simulink model "KinarmSimonTask_260119"  (R2019b)
settings: Solver=ode4  StartTime=0.0  StopTime=inf  FixedStep=BKIN_STEP_TIME  RelTol=1e-3  EnableMultiTasking=on
StartFcn:
  |  warndlg('Dexterit-E models cannot run under simulation. Please compile your model and run it from within Dexterit-E.');set_param(bdroot,'SimulationCommand','stop')
model workspace (MAT data in the model file):
  BKIN_KINEMATIC_FRAME_SIZE = 400
  BKIN_STEP_TIME = 0.00025
  E_COL_LSTIM = 8
  E_COL_RSTIM = 9
  E_CONG = 16
  E_CORRECT = 22
  E_FALSE_START = 28
  E_FIX_OFF = 11
  E_FIX_ON = 31
  E_INCONG = 17
  E_INCORRECT = 24
  E_LEFT_REACHED = 1
  E_LOC_LSIDE = 5
  E_LOC_NEUT = 7
  E_LOC_RSIDE = 6
  E_NEUTRAL = 10
  E_NO_EVENT = 0
  E_RIGHT_REACHED = 2
  E_STIM_OFF = 13
  E_STIM_ON = 12
  E_TIMED_OUT = 29
  E_TRIAL_END = 30
  E_TRIAL_START = 3
  E_WALLS_ON = 4
  FIX_OFF_TIME = 12
  FIX_ON_TIME = 11
  FIX_RAND = 13
  FIX_TARG_COL = 9
  FLICKER_ON = 9
  FLICKER_TIME = 10
  IMAGE_1 = 6
  IMAGE_2 = 7
  INST_TARG_COL = 1
  LBARR_TARG_COL = 4
  LENGTH = 3
  LOAD_X = 1
  LOAD_Y = 2
  LWALL_TARG_COL = 3
  NEUT_ON = 8
  PERTURB_SET = 10
  POSTRESP_DELAY = 4
  RADIUS_VIS = 3
  RBARR_TARG_COL = 6
  REACH_DELAY = 1
  REACH_RAND = 2
  REACH_TO = 3
  RESULT_TARG_COL = 8
  RWALL_TARG_COL = 5
  SPRING_CONST = 5
  START_BLOCK = 14
  START_TARG_COL = 2
  STIM_DIST = 6
  STIM_TARG_COL = 7
  STROKE_WIDTH = 10
  TARG_LENGTH = 3
  TARG_WIDTH = 4
  TEXT = 8
  TEXT_SIZE = 9
  WALL_SHAKE_TOGGLE = 7
  WIDTH = 4
  Width = 4
  X_LENGTH = 4
  Y_LENGTH = 5
  col_x = 1
  col_y = 2
undefined symbols (not defined in the file or in its folder): slselsubs
libraries: Video x11, General x3, KINARM_general x3, KINARM_EP_loads x2
settings Model: ModifiedComment=chris -- Wed Feb 16 09:18:30 2005 -- Version 1.1384  ModifiedHistory=Feb 16/05 - Add error repeat, add offset ramp  ExtModeArmWhenConnect=off  ExtModeLogAll=off  OrderedModelArguments=off  Creator=Chris Grebeldinger  LastModifiedBy=apark2
settings SolverCC: AutoInsertRateTranBlk=on
settings DataIOCC: SaveFormat=Array  SignalLoggingSaveFormat=ModelDataLogs  SaveOutput=off  SaveTime=off  ReturnWorkspaceOutputs=off  SignalLoggingName=sigsOut
settings OptimizationCC: BlockReduction=off  BooleanDataType=off  OptimizeBlockIOStorage=off  BufferReuse=off  GlobalBufferReuse=off  ExpressionFolding=off  ExpressionDepthLimit=2147483647  LocalBlockOutputs=off  InitFltsAndDblsToZero=on  LifeSpan=inf  OptimizeDataStoreBuffers=off  BusAssignmentInplaceUpdate=off
settings DebuggingCC: SaveWithParameterizedLinksMsg=none  UnderspecifiedInitializationDetection=Classic  MergeDetectMultiDrivingBlocksExec=none  SignalResolutionControl=TryResolveAllWithWarning  MultiTaskDSMMsg=warning  FcnCallInpInsideContextMsg=warning  BusObjectLabelMismatch=none  StateNameClashWarn=warning  StrictBusMsg=ErrorOnBusTreatedAsVector  SFUnexpectedBacktrackingDiag=warning  SFNoUnconditionalDefaultTransitionDiag=warning  SFExecutionAtInitializationDiag=none  ArithmeticOperatorsInVariantConditions=warning
settings HardwareCC: ProdBitPerPointer=32  ProdBitPerSizeT=32  ProdBitPerPtrDiffT=32  ProdLargestAtomicFloat=None  ProdWordSize=32  ProdLongLongMode=on  ProdHWDeviceType=Generic->32-bit x86 compatible  TargetLongLongMode=on  TargetIntDivRoundTo=Zero  TargetEndianess=LittleEndian  TargetHWDeviceType=Generic->32-bit x86 compatible
settings ModelReferenceCC: PropagateSignalLabelsOutOfModel=off
settings SFSimCC: SimCustomHeaderCode="#include \"stdlib.h\""  SimUseLocalCustomCode=off  SimParseCustomCode=off  CustomCodeUndefinedFunction=UseInterfaceOnly
settings RTWCC: Description=Simulink Real-Time  SystemTargetFile=slrt.tlc  TemplateMakefile=slrt_default_tmf  RTWUseLocalCustomCode=off  CustomSourceCode="#include \"stdlib.h\""  CodeExecutionProfiling=on
settings CodeAppCC: MaxIdLength=63  StateflowObjectComments=on
settings SimulinkRealTimeCC: TargetFcnLib=ansi_tfl_tmw.mat  GeneratePreprocessorConditionals=Disable all  PreserveStateflowLocalDataDimensions=off
settings ConfigComp: CovMetricSettings=dw  CovHtmlReporting=on  CovSaveCumulativeToWorkspaceVar=on  CovSaveSingleToWorkspaceVar=on  CovExternalEMLEnable=off

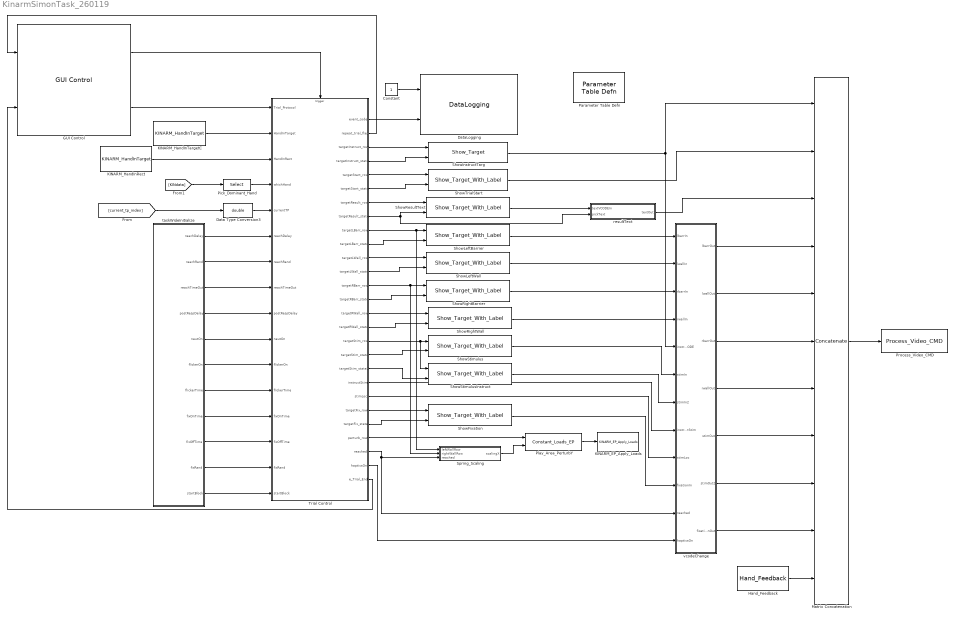
== system KinarmSimonTask_260119 ==
  Constant : Constant
  Data Type Conversion3 : DataTypeConversion  OutDataTypeStr=double
  DataLogging : General/DataLogging  log_event_codes=on  log_analog_inputs=off  show_time_remaining=off  ecat_include=on
  GUI Control : General/GUI Control  task_version=1.0  show_repeat_trial_flag=on  use_custom_tp=off  target_type_str=Circle  Target_Type=1  XYcols=[1 2]  Vcols=3  Lcols=4  indices_padding=[0 0 0 0;0 0 0 0]  target_table_rows=64  load_table_rows=20  tp_table_rows=100
  Hand_Feedback : KINARM_general/Hand_Feedback  feedback_cntl_src=none
  KINARM_EP_Apply_Loads : KINARM_EP_loads/KINARM_EP_Apply_Loads  up_duration=1500  down_duration=1500  max_force=20
  KINARM_HandInRect : KINARM_general/KINARM_HandInTarget  use_dominant_hand=on  target_type=Rectangle  num_states=1  attribcol1=[X_LENGTH Y_LENGTH 0]  attribcol2=[0 0 0]  attribcol3=[0 0 0]  attribcol4=[0 0 0]  attribcol5=[0 0 0]
  KINARM_HandInTargetC : KINARM_general/KINARM_HandInTarget  use_dominant_hand=on  target_type=Circle  num_states=1  attribcol1=[RADIUS_VIS]  attribcol2=[0]  attribcol3=[0]  attribcol4=[0]  attribcol5=[0]
  Matrix Concatenation : Concatenate  NumInputs=11  Mode=Multidimensional array
  Parameter Table Defn : General/Parameter Table Defn  ShowInLibBrowser=0
  Pick_Dominant_Hand : Selector  NumberOfDimensions=2  InputPortWidth=3  IndexOptions=Index vector (dialog),Index vector (dialog)  Indices=[3],[1]  OutputSizes=slselsubs([(-2),(-2)],1),slselsubs([(-2),(-2)],2)
  Play_Area_PerturbY : KINARM_EP_loads/Constant_Loads_EP  use_dom_hand=on  loadcol=[LOAD_X LOAD_Y]  source=port  scaling=1  use_LH_coord=on
  Process_Video_CMD : Video/Process_Video_CMD  video_delay=50
  ShowFixation : Video/Show_Target_With_Label  target_type=Rectangle  num_states=1  attribcol1=[0 0 0 0 0 0 TEXT IMAGE_1 TEXT_SIZE]  attribcol2=[0 0 0 0 0 0 0 0 0]  attribcol3=[0 0 0 0 0 0 0 0 0]  attribcol4=[0 0 0 0 0 0 0 0 0]  attribcol5=[0 0 0 0 0 0 0 0 0]  stateindices_padding=[0 0;0 0;0 0;0 0;0 0]  source=dialog  opacity=100  target_display=Both subject and operator displays
  ShowInstructTarg : Video/Show_Target  target_type=Rectangle  num_states=1  attribcol1=[IMAGE_1 0 0 X_LENGTH Y_LENGTH 0]  attribcol2=[0 0 0 0 0 0]  attribcol3=[0 0 0 0 0 0]  attribcol4=[0 0 0 0 0 0]  attribcol5=[0 0 0 0 0 0]  stateindices_padding=[0 0 0 0 0;0 0 0 0 0;0 0 0 0 0;0 0 0 0 0;0 0 0 0 0]  source=dialog  opacity=100  target_display=Both subject and operator displays  num_col=6
  ShowLeftBarrier : Video/Show_Target_With_Label  target_type=Rectangle  num_states=1  attribcol1=[IMAGE_1 0 0 X_LENGTH Y_LENGTH 0 0 0 0]  attribcol2=[0 0 0 0 0 0 0 0 0]  attribcol3=[0 0 0 0 0 0 0 0 0]  attribcol4=[0 0 0 0 0 0 0 0 0]  attribcol5=[0 0 0 0 0 0 0 0 0]  stateindices_padding=[0 0;0 0;0 0;0 0;0 0]  source=dialog  opacity=100  target_display=Both subject and operator displays
  ShowLeftWall : Video/Show_Target_With_Label  target_type=Rectangle  num_states=2  attribcol1=[IMAGE_1 0 0 X_LENGTH Y_LENGTH 0 0 0 0]  attribcol2=[IMAGE_2 0 0 X_LENGTH Y_LENGTH 0 0 0 0]  attribcol3=[0 0 0 0 0 0 0 0 0]  attribcol4=[0 0 0 0 0 0 0 0 0]  attribcol5=[0 0 0 0 0 0 0 0 0]  stateindices_padding=[0 0;0 0;0 0;0 0;0 0]  source=dialog  opacity=100  target_display=Both subject and operator displays
  ShowResultText : Video/Show_Target_With_Label  target_type=Circle  num_states=4  attribcol1=[0 0 0 0 TEXT IMAGE_2 TEXT_SIZE]  attribcol2=[0 0 0 0 TEXT IMAGE_1 TEXT_SIZE]  attribcol3=[0 0 0 0 TEXT IMAGE_1 TEXT_SIZE]  attribcol4=[0 0 0 0 TEXT IMAGE_1 TEXT_SIZE]  attribcol5=[0 0 0 0 0 0 0]  stateindices_padding=[0 0 0 0;0 0 0 0;0 0 0 0;0 0 0 0;0 0 0 0]  source=dialog  opacity=100  target_display=Both subject and operator displays
  ShowRightBarrier : Video/Show_Target_With_Label  target_type=Rectangle  num_states=1  attribcol1=[IMAGE_1 0 0 X_LENGTH Y_LENGTH 0 0 0 0]  attribcol2=[0 0 0 0 0 0 0 0 0]  attribcol3=[0 0 0 0 0 0 0 0 0]  attribcol4=[0 0 0 0 0 0 0 0 0]  attribcol5=[0 0 0 0 0 0 0 0 0]  stateindices_padding=[0 0;0 0;0 0;0 0;0 0]  source=dialog  opacity=100  target_display=Both subject and operator displays
  ShowRightWall : Video/Show_Target_With_Label  target_type=Rectangle  num_states=2  attribcol1=[IMAGE_1 0 0 X_LENGTH Y_LENGTH 0 0 0 0]  attribcol2=[IMAGE_2 0 0 X_LENGTH Y_LENGTH 0 0 0 0]  attribcol3=[0 0 0 0 0 0 0 0 0]  attribcol4=[0 0 0 0 0 0 0 0 0]  attribcol5=[0 0 0 0 0 0 0 0 0]  stateindices_padding=[0 0;0 0;0 0;0 0;0 0]  source=dialog  opacity=100  target_display=Both subject and operator displays
  ShowStimulus : Video/Show_Target_With_Label  target_type=Rectangle  num_states=2  attribcol1=[IMAGE_1 0 0 X_LENGTH Y_LENGTH 0 0 0 0]  attribcol2=[IMAGE_2 0 0 X_LENGTH Y_LENGTH 0 0 0 0]  attribcol3=[0 0 0 0 0 0 0 0 0]  attribcol4=[0 0 0 0 0 0 0 0 0]  attribcol5=[0 0 0 0 0 0 0 0 0]  stateindices_padding=[0 0;0 0;0 0;0 0;0 0]  source=dialog  opacity=100  target_display=Both subject and operator displays
  ShowStimulusInstruct : Video/Show_Target_With_Label  target_type=Rectangle  num_states=2  attribcol1=[IMAGE_1 0 0 X_LENGTH Y_LENGTH 0 0 0 0]  attribcol2=[IMAGE_2 0 0 X_LENGTH Y_LENGTH 0 0 0 0]  attribcol3=[0 0 0 0 0 0 0 0 0]  attribcol4=[0 0 0 0 0 0 0 0 0]  attribcol5=[0 0 0 0 0 0 0 0 0]  stateindices_padding=[0 0;0 0;0 0;0 0;0 0]  source=dialog  opacity=100  target_display=Both subject and operator displays
  ShowTrialStart : Video/Show_Target_With_Label  target_type=Circle  num_states=1  attribcol1=[IMAGE_1 IMAGE_2 STROKE_WIDTH RADIUS_VIS 0 0 0]  attribcol2=[0 0 0 0 0 0 0]  attribcol3=[0 0 0 0 0 0 0]  attribcol4=[0 0 0 0 0 0 0]  attribcol5=[0 0 0 0 0 0 0]  stateindices_padding=[0 0 0 0;0 0 0 0;0 0 0 0;0 0 0 0;0 0 0 0]  source=dialog  opacity=100  target_display=Both subject and operator displays
  Spring_Scaling : Subsystem
  Trial Control : Stateflow chart  TreatAsAtomicUnit=on
  resultText : Subsystem
  taskWideInitialize : Subsystem
  vcodeChange : Subsystem
  wires:
  Trial Control/27(e_Trial_End) -> GUI Control/2
  Matrix Concatenation/1 -> Process_Video_CMD/1
  Trial Control/1(event_code) -> DataLogging/2
  Constant/1 -> DataLogging/1
  GUI Control/2 -> Trial Control/1(Trial_Protocol)
  Trial Control/2(repeat_trial_flag) -> GUI Control/1
  [current_tp_index] -> Data Type Conversion3/1
  ShowResultText/1 -> resultText/1(textVCODEIn)
  KINARM_HandInTargetC/1 -> Trial Control/2(HandInTarget)
  GUI Control/1 -> Trial Control/Trigger
  Data Type Conversion3/1 -> Trial Control/5(currentTP)
  Trial Control/15(targetRWall_row) -> ShowRightWall/1
  Trial Control/11(targetLWall_row) -> ShowLeftWall/1
  Trial Control/12(targetLWall_state) -> ShowLeftWall/2
  Trial Control/7(targetResult_row) -> ShowResultText/1
  Trial Control/8(targetResult_state) -> ShowResultText/2, resultText/2(pickText)
  taskWideInitialize/1(reachDelay) -> Trial Control/6(reachDelay)
  taskWideInitialize/4(postRespDelay) -> Trial Control/9(postRespDelay)
  Trial Control/16(targetRWall_state) -> ShowRightWall/2
  resultText/1(textOut) -> Matrix Concatenation/3
  Trial Control/3(targetInstruct_row) -> ShowInstructTarg/1
  Trial Control/4(targetInstruct_state) -> ShowInstructTarg/2
  ShowInstructTarg/1 -> vcodeChange/5(instructVCODE), Matrix Concatenation/1
  Play_Area_PerturbY/1 -> KINARM_EP_Apply_Loads/1
  Trial Control/26(hapticsOn) -> vcodeChange/12(hapticsOn)
  Trial Control/24(perturb_row) -> Play_Area_PerturbY/1
  Trial Control/5(targetStart_row) -> ShowTrialStart/1
  Trial Control/6(targetStart_state) -> ShowTrialStart/2
  ShowTrialStart/1 -> Matrix Concatenation/2
  taskWideInitialize/3(reachTimeOut) -> Trial Control/8(reachTimeOut)
  Trial Control/25(reached) -> vcodeChange/11(reached), Spring_Scaling/3(reached)
  ShowLeftWall/1 -> vcodeChange/2(lwallIn)
  ShowRightWall/1 -> vcodeChange/4(rwallIn)
  vcodeChange/2(lwallOut) -> Matrix Concatenation/5
  vcodeChange/4(rwallOut) -> Matrix Concatenation/7
  KINARM_HandInRect/1 -> Trial Control/3(HandInRect)
  vcodeChange/5(stimOut) -> Matrix Concatenation/8
  Hand_Feedback/1 -> Matrix Concatenation/11
  Spring_Scaling/1(scalingX) -> Play_Area_PerturbY/2
  [KINdata] -> Pick_Dominant_Hand/1
  Pick_Dominant_Hand/1 -> Trial Control/4(whichHand)
  Trial Control/9(targetLBarr_row) -> ShowLeftBarrier/1, Spring_Scaling/1(leftWallRow)
  Trial Control/10(targetLBarr_state) -> ShowLeftBarrier/2
  ShowLeftBarrier/1 -> vcodeChange/1(lbarrIn)
  Trial Control/13(targetRBarr_row) -> Spring_Scaling/2(rightWallRow), ShowRightBarrier/1
  Trial Control/14(targetRBarr_state) -> ShowRightBarrier/2
  ShowRightBarrier/1 -> vcodeChange/3(rbarrIn)
  vcodeChange/1(lbarrOut) -> Matrix Concatenation/4
  vcodeChange/3(rbarrOut) -> Matrix Concatenation/6
  taskWideInitialize/5(neutOn) -> Trial Control/10(neutOn)
  Trial Control/17(targetStim_row) -> ShowStimulusInstruct/1, ShowStimulus/1
  Trial Control/18(targetStim_state) -> ShowStimulus/2
  ShowStimulus/1 -> vcodeChange/6(stimIn)
  Trial Control/21(stimLoc) -> vcodeChange/9(stimLoc)
  taskWideInitialize/2(reachRand) -> Trial Control/7(reachRand)
  taskWideInitialize/6(flickerOn) -> Trial Control/11(flickerOn)
  taskWideInitialize/7(flickerTime) -> Trial Control/12(flickerTime)
  ShowFixation/1 -> vcodeChange/10(fixationIn)
  Trial Control/22(targetFix_row) -> ShowFixation/1
  Trial Control/23(targetFix_state) -> ShowFixation/2
  vcodeChange/7("fixationOut ") -> Matrix Concatenation/10
  taskWideInitialize/9(fixOffTime) -> Trial Control/14(fixOffTime)
  taskWideInitialize/10(fixRand) -> Trial Control/15(fixRand)
  taskWideInitialize/8(fixOnTime) -> Trial Control/13(fixOnTime)
  Trial Control/20(instructStim) -> vcodeChange/8(instructStim)
  vcodeChange/6(stimOut2) -> Matrix Concatenation/9
  ShowStimulusInstruct/1 -> vcodeChange/7("stimIn2 ")
  Trial Control/19(targetStim_state2) -> ShowStimulusInstruct/2
  taskWideInitialize/11(startBlock) -> Trial Control/16(startBlock)

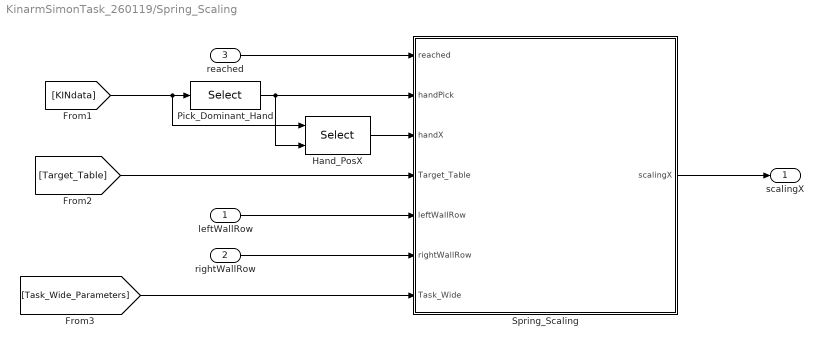
== system KinarmSimonTask_260119/Spring_Scaling ==
  leftWallRow : Inport
  rightWallRow : Inport  Port=2
  reached : Inport  Port=3
  Hand_PosX : Selector  NumberOfDimensions=2  InputPortWidth=3  IndexOptions=Index vector (port),Index vector (dialog)  Indices=[3],[23]  OutputSizes=slselsubs([(-2),(-2)],1),slselsubs([(-2),(-2)],2)
  Pick_Dominant_Hand : Selector  NumberOfDimensions=2  InputPortWidth=3  IndexOptions=Index vector (dialog),Index vector (dialog)  Indices=[3],[1]  OutputSizes=slselsubs([(-2),(-2)],1),slselsubs([(-2),(-2)],2)
  Spring_Scaling : MATLAB Function  TreatAsAtomicUnit=on
  scalingX : Outport  VectorParamsAs1DForOutWhenUnconnected=off
  wires:
  Spring_Scaling/1(scalingX) -> scalingX/1
  reached/1 -> Spring_Scaling/1(reached)
  [Target_Table] -> Spring_Scaling/4(Target_Table)
  [KINdata] -> Hand_PosX/1, Pick_Dominant_Hand/1
  Pick_Dominant_Hand/1 -> Hand_PosX/2, Spring_Scaling/2(handPick)
  Hand_PosX/1 -> Spring_Scaling/3(handX)
  [Task_Wide_Parameters] -> Spring_Scaling/7(Task_Wide)
  leftWallRow/1 -> Spring_Scaling/5(leftWallRow)
  rightWallRow/1 -> Spring_Scaling/6(rightWallRow)

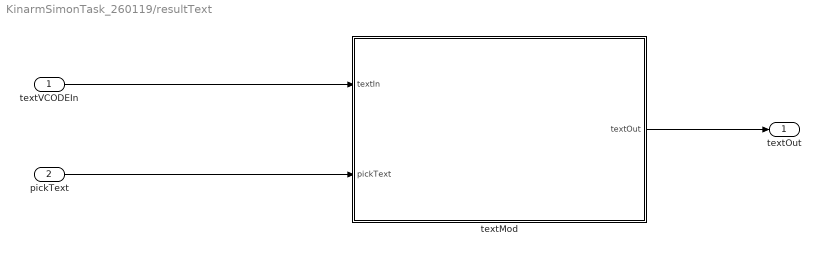
== system KinarmSimonTask_260119/resultText ==
  textVCODEIn : Inport
  pickText : Inport  Port=2
  textMod : MATLAB Function  TreatAsAtomicUnit=on
  textOut : Outport
  wires:
  textMod/1(textOut) -> textOut/1
  textVCODEIn/1 -> textMod/1(textIn)
  pickText/1 -> textMod/2(pickText)

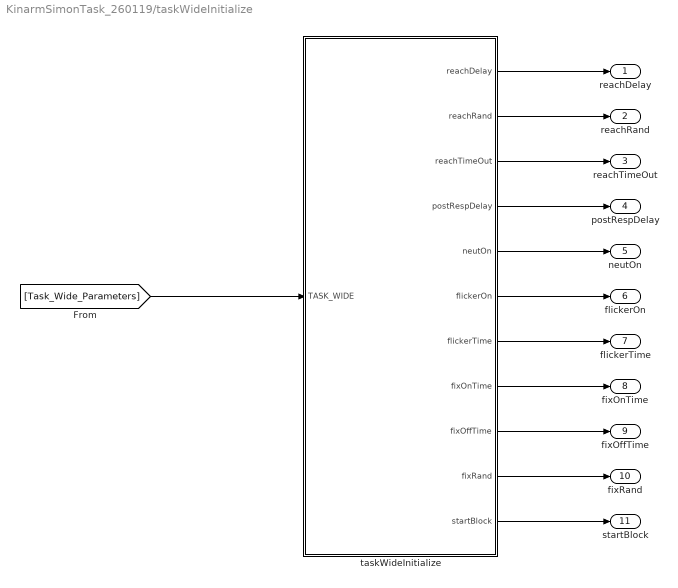
== system KinarmSimonTask_260119/taskWideInitialize ==
  taskWideInitialize : MATLAB Function  TreatAsAtomicUnit=on
  reachDelay : Outport
  reachRand : Outport  Port=2
  reachTimeOut : Outport  Port=3
  postRespDelay : Outport  Port=4
  neutOn : Outport  Port=5
  flickerOn : Outport  Port=6
  flickerTime : Outport  Port=7
  fixOnTime : Outport  Port=8
  fixOffTime : Outport  Port=9
  fixRand : Outport  Port=10
  startBlock : Outport  Port=11
  wires:
  [Task_Wide_Parameters] -> taskWideInitialize/1(TASK_WIDE)
  taskWideInitialize/1(reachDelay) -> reachDelay/1
  taskWideInitialize/3(reachTimeOut) -> reachTimeOut/1
  taskWideInitialize/4(postRespDelay) -> postRespDelay/1
  taskWideInitialize/5(neutOn) -> neutOn/1
  taskWideInitialize/2(reachRand) -> reachRand/1
  taskWideInitialize/7(flickerTime) -> flickerTime/1
  taskWideInitialize/6(flickerOn) -> flickerOn/1
  taskWideInitialize/9(fixOffTime) -> fixOffTime/1
  taskWideInitialize/10(fixRand) -> fixRand/1
  taskWideInitialize/8(fixOnTime) -> fixOnTime/1
  taskWideInitialize/11(startBlock) -> startBlock/1

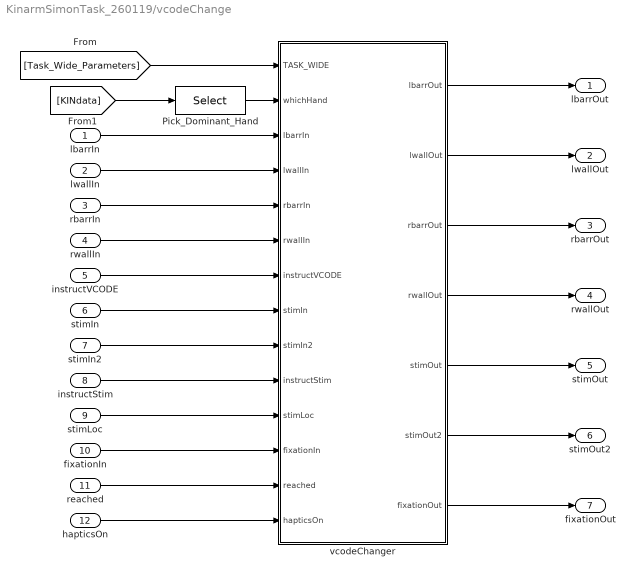
== system KinarmSimonTask_260119/vcodeChange ==
  lbarrIn : Inport
  lwallIn : Inport  Port=2
  rbarrIn : Inport  Port=3
  rwallIn : Inport  Port=4
  instructVCODE : Inport  Port=5
  stimIn : Inport  Port=6
  "stimIn2 " : Inport  Port=7
  instructStim : Inport  Port=8
  stimLoc : Inport  Port=9
  fixationIn : Inport  Port=10
  reached : Inport  Port=11
  hapticsOn : Inport  Port=12
  Pick_Dominant_Hand : Selector  NumberOfDimensions=2  InputPortWidth=3  IndexOptions=Index vector (dialog),Index vector (dialog)  Indices=[3],[1]  OutputSizes=slselsubs([(-2),(-2)],1),slselsubs([(-2),(-2)],2)
  "vcodeChanger " : MATLAB Function  TreatAsAtomicUnit=on
  lbarrOut : Outport
  lwallOut : Outport  Port=2
  rbarrOut : Outport  Port=3
  rwallOut : Outport  Port=4
  stimOut : Outport  Port=5
  stimOut2 : Outport  Port=6
  "fixationOut " : Outport  Port=7
  wires:
  hapticsOn/1 -> "vcodeChanger "/14(hapticsOn)
  reached/1 -> "vcodeChanger "/13(reached)
  [Task_Wide_Parameters] -> "vcodeChanger "/1(TASK_WIDE)
  lwallIn/1 -> "vcodeChanger "/4(lwallIn)
  rwallIn/1 -> "vcodeChanger "/6(rwallIn)
  "vcodeChanger "/2(lwallOut) -> lwallOut/1
  "vcodeChanger "/4(rwallOut) -> rwallOut/1
  "vcodeChanger "/5(stimOut) -> stimOut/1
  stimIn/1 -> "vcodeChanger "/8(stimIn)
  [KINdata] -> Pick_Dominant_Hand/1
  Pick_Dominant_Hand/1 -> "vcodeChanger "/2(whichHand)
  rbarrIn/1 -> "vcodeChanger "/5(rbarrIn)
  lbarrIn/1 -> "vcodeChanger "/3(lbarrIn)
  "vcodeChanger "/1(lbarrOut) -> lbarrOut/1
  "vcodeChanger "/3(rbarrOut) -> rbarrOut/1
  stimLoc/1 -> "vcodeChanger "/11(stimLoc)
  fixationIn/1 -> "vcodeChanger "/12(fixationIn)
  "vcodeChanger "/7(fixationOut) -> "fixationOut "/1
  instructVCODE/1 -> "vcodeChanger "/7(instructVCODE)
  instructStim/1 -> "vcodeChanger "/10(instructStim)
  "vcodeChanger "/6(stimOut2) -> stimOut2/1
  "stimIn2 "/1 -> "vcodeChanger "/9(stimIn2)

== matlab function KinarmSimonTask_260119/vcodeChange/vcodeChanger  ==
  data: lbarrOut output; lwallOut output; rbarrOut output; rwallOut output; stimOut output; stimOut2 output; TASK_WIDE input; whichHand input; lbarrIn input; lwallIn input; rbarrIn input; rwallIn input; instructVCODE input; stimIn input; stimIn2 input; instructStim input; stimLoc input; fixationIn input; reached input; hapticsOn input; BKIN_STEP_TIME parameter; WALL_SHAKE_TOGGLE parameter; STIM_DIST parameter; fixationOut output
function [lbarrOut, lwallOut, rbarrOut, rwallOut, stimOut, stimOut2, fixationOut] =...
    fcn(TASK_WIDE, whichHand, lbarrIn, lwallIn, rbarrIn, rwallIn, instructVCODE, stimIn, stimIn2, instructStim, stimLoc, fixationIn, reached, hapticsOn, BKIN_STEP_TIME, WALL_SHAKE_TOGGLE, STIM_DIST)
%this function shakes the Walls and places the Stimulus in the appropriate
%location
%some vcode are routed through to make things look nicer

%initialize taskwides
shakeOnOff = TASK_WIDE(WALL_SHAKE_TOGGLE); %turn on (1) or off (0) Wall shaking feature
stimDist = TASK_WIDE(STIM_DIST)/100; %get the distance the Stimulus should move
dt = BKIN_STEP_TIME;
shakeScalar = 1/8; %speed of Wall shake
shakeLim = 0.01; %distance of shaking

%set output vcodes
stimOut = stimIn; %stimulus vcode
stimOut2 = stimIn2; %stimulus vcode which is only used to show the state of the right movement stimulus - turned off otherwise
fixationOut = fixationIn; %fixation cross vcode
if (whichHand == 2) %if the left hand is used
    lbarrOut = rbarrIn; %flip Barrier
    lwallOut = rwallIn;
    rbarrOut = lbarrIn;
    rwallOut = lwallIn;
    if (stimLoc == 1) %if Stimulus on the left (make it go on the right)
        stimOut(1,3) = stimIn(1,3) + stimDist;
    elseif (stimLoc == 2) %if Stimulus on the right (make it go on the left)
        stimOut(1,3) = stimIn(1,3) - stimDist;
    end
else %right hand used
    lbarrOut = lbarrIn;
    lwallOut = lwallIn;
    rbarrOut = rbarrIn;
    rwallOut = rwallIn;
    if (stimLoc == 1) %Stim on left
        stimOut(1,3) = stimIn(1,3) - stimDist;
    elseif (stimLoc == 2) %Stim on right
        stimOut(1,3) = stimIn(1,3) + stimDist;
    end
end

if (instructStim == 1) %turn on 2 stimulus targets for instruction purposes
    stimOut(3) = instructVCODE(3)-stimOut(10)*1.5; %adjust position of stimulus based on instruction area
    stimOut(4) = instructVCODE(4);
    stimOut2(3) = instructVCODE(3)+stimOut(10)*1.5;
    stimOut2(4) = instructVCODE(4);
end

%set up Wall shaking
persistent atTime0 shakeWall
if (isempty(atTime0))
    atTime0 = 0;
    shakeWall = 0;
end

if (hapticsOn == 1) %if reached successfully
    if (reached == 1) %if left Wall reached successfully
        if (shakeWall <= shakeLim && shakeOnOff == 1) %if wallshake is on
            shakeWall = shakeWall + dt*shakeScalar; %increase shake
        else
            shakeWall = 0;
        end
        lwallOut(1,3) = lwallOut(1,3)-shakeWall; %left Wall shake
    elseif (reached == 2) %if right Wall reached successfully
        if (shakeWall <= shakeLim && shakeOnOff == 1)
            shakeWall = shakeWall + dt*shakeScalar; %increase shake
        else
            shakeWall = 0;
        end
        rwallOut(1,3) = rwallOut(1,3)+shakeWall;
    end
end

if (reached == 0) %reset the shaking (probably dont need any more)
    atTime0 = [];
end

== stateflow chart KinarmSimonTask_260119/Trial Control ==
  state Initialize/
    %setup the variables
    targetInstruct_row = Trial_Protocol(INST_TARG_COL); %Instruction Image shown to participants
    targetStart_row = Trial_Protocol(START_TARG_COL); %target for hand in to start task
    targetResult_row = Trial_Protocol(RESULT_TARG_COL); %result text target
    targetLBarr_row = Trial_Protocol(LBARR_TARG_COL); %left physical Barrier
    targetLWall_row = Trial_Protocol(LWALL_TARG_COL); %show left virtual Wall
    targetRBarr_row = Trial_Protocol(RBARR_TARG_COL); %right physical Barrier
    targetRWall_row = Trial_Protocol(RWALL_TARG_COL); %show right virtual Wall
    targetStim_row = Trial_Protocol(STIM_TARG_COL); %show Stimulus
    targetFix_row = Trial_Protocol(FIX_TARG_COL); %show Fixation Cross
    targetInstruct_state = 0; %turn off Instruction Image
    targetStart_state = 0; %turn off Start Target
    targetResult_state = 0; %turn off Result Target
    targetLBarr_state = 0; %turn off left Barrier
    targetLWall_state = 0; %turn off left Wall
    targetRBarr_state = 0; %turn off right Barrier
    targetRWall_state = 0; %turn off right Wall
    targetStim_state = 0; %turn off Stimulus
    targetStim_state2 = 0; %turn off instruction stimulus
    targetFix_state = 0; %turn off Fixation Cross
    hapticsOn = 0; %no haptic feedback
    reached = 0; %outputs the Wall reached (1 = left, 2 = right)
    instructStim = 0; %flag for turning on the 2nd stimulus target only used for the instruction image
  state MainTrial
    state checkHandOut/
      state wallsAppear/
        %turn on Walls
        targetLBarr_state = 1;
        targetLWall_state = 1;
        targetRBarr_state = 1;
        targetRWall_state = 1;
        event_code = E_WALLS_ON;
      state fixationOn/
        %turn on fixation cross
        targetFix_state = 1;
        event_code = E_FIX_ON;
      state fixationOff/
        %turn off fixation cross for a time
        targetFix_state = 0;
        event_code = E_FIX_OFF;
      wallsAppear -> fixationOn : %holding delay+random
          | after(reachDelay+randReach,msec)
      fixationOn -> fixationOff : after(fixOnTime,msec)
    state showInstruction/
      %show Instruction Image, Start
      %Target, and stimuli for left and
      %right reaching
      targetInstruct_state = 1;
      targetStim_state = 1;
      targetStim_state2 = 2;
      instructStim = 1;
      targetStart_state = 1;
      targetResult_state = 1;
    state startTrial/
      %turn on Start Target, get perturbation direction, Stimulus location and colour
      entry:
      targetInstruct_state = 0; %turn off Instruct Image
      targetStart_state = 1; %turn on Start Target
      perturb_row = Trial_Protocol(PERTURB_SET); %get the perturbation
      [stimLoc,stimCol] = pickSimon(currentTP,neutOn); %get Stimulus location and colour
      targetResult_state = 0;
      randReach = reachRand*rand();
      randFix = fixRand*rand();
      targetStim_state = 0;
      targetStim_state2 = 0;
      instructStim = 0;
      event_code = E_TRIAL_START;
    state reset/
      %turn on the start targ
      %and turn off the result
      targetStart_state = 1;
      targetResult_state = 0;
    state handStart/
      %wait for participant
      %to see instruction
    state falseStart/
      %left Start Target too early
      event_code = E_FALSE_START;
      targetResult_state = 4;
      targetFix_state = 0;
    state stimColourEvents/
      %Stimulus colour event codes
      state moveLeft/
        event_code = E_COL_LSTIM;
      state moveRight/
        event_code = E_COL_RSTIM;
    state nice3/
    state stimLocEvents/
      %event codes for Stimulus location
      state stimOnLeft/
        event_code = E_LOC_LSIDE;
      state stimOnRight/
        event_code = E_LOC_RSIDE;
      state stimOnMiddle/
        event_code = E_LOC_NEUT;
    state trialEvents/
      %event codes for trial type
      state neutral/
        event_code = E_NEUTRAL;
      state incong/
        event_code = E_INCONG;
      state cong/
        event_code = E_CONG;
    state nice2/
    state nice1/
      %just looks nice
    state stimAppear/
      %turn off show Stimulus
      targetStim_state = stimCol;
      targetStart_state = 0;
      event_code = E_STIM_ON;
      simonCong = mod(stimCol+stimLoc,2);
    state nice4/
    state leftReach/
      %left Wall reached
      event_code = E_LEFT_REACHED;
    state resultEvent/
      %send out result event
      state correct/
        %reach was correct and
        %turn on haptic feedback
        hapticsOn = 1;
        event_code = E_CORRECT;
      state timeoutTrial/
        %didnt reach a Wall
        event_code = E_TIMED_OUT;
        targetResult_state = 3;
        targetStart_state = 0;
      state incorrect/
        %reach was incorrect and show
        %text on screen
        event_code = E_INCORRECT;
        targetResult_state = 2;
    state leftCorrect/
      %left correct
      reached = 1;
    state stimulusOff/
      %turn off Stimulus
      %when flickerOn = 1
      event_code = E_STIM_OFF;
      targetStim_state = 0;
    state rightReach/
      %right Wall reached
      event_code = E_RIGHT_REACHED;
    state rightCorrect/
      %right correct
      reached = 2;
    state trialEnd/
      %turn off all targets
      event_code = E_TRIAL_END;
      hapticsOn = 0;
      reached = 0;
      targetInstruct_state = 0;
      targetStart_state = 0;
      targetResult_state = 0;
      targetLBarr_state = 0;
      targetLWall_state = 0;
      targetRBarr_state = 0;
      targetRWall_state = 0;
      targetStim_state = 0;
    state rightReachWrong/
      %turn off reached incorrect Wall
      targetRWall_state = 0;
    state leftReachWrong/
      %turn off reached incorrect Wall
      targetLWall_state = 0;
    startTrial -> reset
    reset -> wallsAppear : %check hand in target
        | [HandInTarget(targetStart_row) == 1]
    (junction 841) -> reset : after(postRespDelay/2,msec)
    handStart -> startTrial [order 1] : after(startBlock,msec)
    showInstruction -> handStart : %check hand in target
        | [HandInTarget(targetStart_row) == 1]
    handStart -> showInstruction [order 2] : %hand out
        | [HandInTarget(targetStart_row) == 0]
    checkHandOut -> falseStart : %hand left the start target
        | [HandInTarget(targetStart_row) == 0]
    falseStart -> (junction 841) : %hand back in start
        | [HandInTarget(targetStart_row) == 1]
    nice3 -> moveLeft [order 2] : %move left
        | [stimCol == 1]
    nice2 -> stimOnLeft [order 2] : %Stimulus left side
        | [stimLoc == 1]
    nice1 -> neutral [order 3] : %neutral trial
        | [stimLoc == 3]
    stimLocEvents -> nice3 : after(1,msec)
    nice3 -> moveRight [order 1] : %move right
        | [stimCol == 2]
    trialEvents -> nice2 : after(1,msec)
    stimColourEvents -> (junction 823) [order 1] : %Stimulus flickers
        | [flickerOn == 1]
    stimColourEvents -> (junction 832) [order 2] : %Stimulus doesnt flicker
        | [flickerOn == 0]
    nice1 -> incong [order 2] : %incongruent if not neutral
        | [stimLoc < 3 && simonCong == 1]
    nice2 -> stimOnRight [order 1] : %Stimulus right side
        | [stimLoc == 2]
    fixationOff -> stimAppear : after(fixOffTime+randFix,msec)
    nice1 -> cong [order 1] : %congruent if not neutral
        | [stimLoc < 3 && simonCong == 0]
    nice2 -> stimOnMiddle [order 3] : %Stimulus in middle
        | [stimLoc == 3]
    stimAppear -> nice1 : after(1,msec)
    (junction 832) -> nice4 : after(1,msec)
    (junction 823) -> stimulusOff : after(flickerTime,msec)
    nice4 -> (junction 784) [order 2] : %right hand used
        | [whichHand == 1]
    (junction 784) -> leftReach [order 2] : %right hand in left Wall
        | [HandInRect(targetLBarr_row)==1]
    (junction 784) -> rightReach [order 1] : %right hand in right Wall
        | [HandInRect(targetRBarr_row)==1]
    (junction 785) -> leftReach [order 1] : %left hand in left wall
        | [HandInRect(targetRBarr_row)==1]
    leftReach -> leftCorrect [order 1] : %correctly reached left
        | [stimCol == 1]
    leftReach -> (junction 801) [order 2] : after(1,msec)
    leftCorrect -> correct : after(1,msec)
    rightReach -> rightCorrect [order 1] : %correctly reached right
        | [stimCol == 2]
    rightCorrect -> correct : after(1,msec)
    nice4 -> (junction 785) [order 3] : %left hand used
        | [whichHand == 2]
    (junction 785) -> rightReach [order 2] : %right hand in right wall
        | [HandInRect(targetLBarr_row)==1]
    stimulusOff -> nice4 : after(1,msec)
    rightReach -> (junction 798) [order 2] : after(1,msec)
    nice4 -> timeoutTrial [order 1] : %didnt reach in time
        | after(reachTimeOut,msec)
    (junction 798) -> rightReachWrong [order 1] : [whichHand == 1]
    (junction 798) -> leftReachWrong [order 2] : [whichHand == 2]
    (junction 801) -> rightReachWrong [order 2] : [whichHand == 2]
    rightReachWrong -> incorrect
    (junction 801) -> leftReachWrong [order 1] : [whichHand == 1]
    leftReachWrong -> incorrect
    resultEvent -> trialEnd : %intertrial delay
        | after(postRespDelay,msec)
  state Inter_Trial_State/
    %turn off all targets
    entry:
    event_code = 0;
    repeat_trial_flag = 0;
    hapticsOn = 0;
    reached = 0;
    targetInstruct_state = 0;
    targetStart_state = 0;
    targetResult_state = 0;
    targetLBarr_state = 0;
    targetLWall_state = 0;
    targetRBarr_state = 0;
    targetRWall_state = 0;
    targetStim_state = 0;
    targetFix_state = 0;
    e_Trial_End;
  state RepeatTrial/
    entry:
    repeat_trial_flag = 1;
  (default) -> Initialize
  Initialize -> showInstruction : %wait for task to start
      | [currentTP > 0]
  Inter_Trial_State -> startTrial : after(1,msec)
  RepeatTrial -> Inter_Trial_State : after(1,msec)
  MainTrial -> RepeatTrial : e_ExitTrialNow
      | % e_ExitTrialNow event occurs if the
      | % Dex pause is pressed by the operator
  trialEnd -> Inter_Trial_State : after(1,msec)
  data: locStim function_output; colStim function_output; nowTP function_input; neutIn function_input; event_code output [0..]; repeat_trial_flag output; targetInstruct_row output; targetInstruct_state output; targetStart_row output; targetStart_state output; Trial_Protocol input; HandInTarget input; HandInRect input; whichHand input; targetResult_row output; targetResult_state output; targetLBarr_row output; targetLBarr_state output; targetLWall_row output; targetLWall_state output; targetRBarr_row output; targetRBarr_state output; targetRWall_row output; targetRWall_state output; targetStim_row output; targetStim_state output; targetStim_state2 output; instructStim output; stimLoc output; targetFix_row output; targetFix_state output; perturb_row output; reached output; hapticsOn output; currentTP input; reachDelay input; reachRand input; reachTimeOut input; postRespDelay input; stimCol local; simonCong local; neutOn input; flickerOn input; flickerTime input; fixOnTime input; randReach local; fixOffTime input; fixRand input; randFix local; startBlock input
  events: e_clk input RISING_EDGE_EVENT; e_ExitTrialNow input RISING_EDGE_EVENT; e_Trial_End output EITHER_EDGE_EVENT
  function [locStim,colStim] = pickSimon(nowTP,neutIn):
    | function [locStim,colStim] = pickSimon(nowTP,neutIn)
    | %This function sets up an array for picking the colour associated with left
    | %or right movements (left movement = 1, right movement = 2) and location 
    | %(1 = left side, 2 = right side, 3 = neutral (middle)). Task has
    | %functionality to include or remove neutral trials with the neutIn input
    | %(0 = no neutral trials, 1 = neutral trials).
    | %Neutral included runs need to have at least 6 TP used (2 Stimulus colours 
    | %for left and right movement, 3 locations for Stimulus to appear) and non 
    | %neutral runs need to have at least 4 TP (2 Stimulus colours, 2 locations).
    | 
    | %% set up array to pull distractor and centre arrow states
    | 
    | %location and colour of the Stimulus based on the current TP (all odd
    | %positioned values should be 1 in row 2 (left movements are odd TP, and all 
    | %even should be 2 in row 2 (right movements are even TP))
    | simonNeut = [1 1 2 2 3 3;... %location of Stimulus (1 = left, 2 = right, 3 = neutral)
    |              1 2 1 2 1 2];   %colour of Stimulus (1 = left movement colour, 2 = right movement colour)
    |             
    | simonTight = [1 1 2 2;... %location of Stimulus (1 = left, 2 = right)
    |               1 2 1 2];   %colour of Stimulus (1 = left movement colour, 2 = right movement colour)
    |             
    | %% output variables
    | 
    | if (neutIn == 1) %keep neutral trials
    |     simonArray = simonNeut; %groups of 6 trials in block table MUST
    | else %remove neutral trials if unwanted 
    |     simonArray = simonTight; %groups of 4 trials in block table MUST
    | end
    | 
    | locStim = simonArray(1,nowTP); % pick Stimulus location
    | colStim = simonArray(2,nowTP); % pick Stimulus colour

== matlab function KinarmSimonTask_260119/taskWideInitialize/taskWideInitialize ==
  data: TASK_WIDE input; reachDelay output; reachRand output; reachTimeOut output; postRespDelay output; REACH_DELAY parameter; REACH_TO parameter; POSTRESP_DELAY parameter; NEUT_ON parameter; neutOn output; flickerOn output; flickerTime output; fixOnTime output; REACH_RAND parameter; FLICKER_ON parameter; FLICKER_TIME parameter; fixOffTime output; FIX_OFF_TIME parameter; fixRand output; FIX_RAND parameter; FIX_ON_TIME parameter; startBlock output; START_BLOCK parameter
function [reachDelay, reachRand, reachTimeOut, postRespDelay, neutOn, flickerOn, flickerTime, fixOnTime, fixOffTime, fixRand, startBlock] =...
    fcn(TASK_WIDE, REACH_DELAY, REACH_TO, POSTRESP_DELAY, NEUT_ON, REACH_RAND, FLICKER_ON, FLICKER_TIME, FIX_OFF_TIME, FIX_RAND, FIX_ON_TIME, START_BLOCK)  

%% task wide parameter outputs
reachDelay = TASK_WIDE(REACH_DELAY); %holding in Start Target time
reachRand = TASK_WIDE(REACH_RAND); %random amount of time added to reachDelay
reachTimeOut = TASK_WIDE(REACH_TO); %alloted time for reaching
postRespDelay = TASK_WIDE(POSTRESP_DELAY); %time between trials
neutOn = TASK_WIDE(NEUT_ON); %turn the neutral trials on (1) or off (0)
flickerOn = TASK_WIDE(FLICKER_ON); %have Stimulus turn off quickly (1) or stay on (0)
flickerTime = TASK_WIDE(FLICKER_TIME); %time that the Stimulus stays on if flickerOn = 1
fixOnTime = TASK_WIDE(FIX_ON_TIME); %time that fixation cross turns on for
fixOffTime = TASK_WIDE(FIX_OFF_TIME); %time between fixation cross off and stimulus on
fixRand = TASK_WIDE(FIX_RAND); %random time added to fixOffTime
startBlock = TASK_WIDE(START_BLOCK); %time for participants to hold the start target to begin the task

== matlab function KinarmSimonTask_260119/Spring_Scaling/Spring_Scaling ==
  data: reached input; handPick input; handX input; Target_Table input; leftWallRow input; rightWallRow input; Task_Wide input; SPRING_CONST parameter; scalingX output; X_LENGTH parameter
function scalingX  = Spring_Scaling(reached, handPick, handX, Target_Table, leftWallRow, rightWallRow, Task_Wide, SPRING_CONST, X_LENGTH)
%This function makes the physical Barriers in the task into springs that
%push the hand back

%initialize variables
springConst = Task_Wide(SPRING_CONST)* 10; %10 is a minor adjustment for cm -> m conversion (20 feels good)

%get location of the left and right Barriers
if (handPick == 1) %if right hand
    leftBarrier = Target_Table(leftWallRow,1)*0.01 + Target_Table(leftWallRow,X_LENGTH)*0.005; %centre of Barrier and half of the length is the right side of the left Barrier
    rightBarrier = Target_Table(rightWallRow,1)*0.01 - Target_Table(rightWallRow,X_LENGTH)*0.005; %left side of the right Barrier
else %if left hand
    leftBarrier = Target_Table(rightWallRow,1)*0.01 + Target_Table(rightWallRow,X_LENGTH)*0.005; %left Barrier is now right Barrier 
    rightBarrier = Target_Table(leftWallRow,1)*0.01 - Target_Table(leftWallRow,X_LENGTH)*0.005; %right Barrier is now left Barrier
end

leftCHECK = double(handX < leftBarrier); %check if the hand is in the left Barrier
rightCHECK = double(handX > rightBarrier); %check if the hand is in the right Barrier
    
%% SPRING SCALING 
% set conditions for the scaling to push the hand back into the centre
scalingX = 0;
if (reached == 1) %only start spring scaling once the left Barrier is reached
    if (leftCHECK) %check left Barrier check
        if (handPick == 1) %accounts for flipped left/right hand usage
            scalingX = springConst * (leftBarrier - handX); %scaling based on basic spring force equation f=kx (force = constant*distance)
            if (leftBarrier - handX > 10) %safety
                scalingX = springConst * 10;
            end
        else %flipped scaling to account for left/right hand usage
            scalingX = -springConst * (leftBarrier - handX);
            if (leftBarrier - handX > 10) %safety
                scalingX = -springConst * 10;
            end
        end
    else
        scalingX = 0;
    end
end

if (reached == 2) %if hand is in the right Barrier
    if (rightCHECK) %check right boundary condition
        if (handPick == 1) %right hand use
            scalingX = -springConst * (rightBarrier - handX);
            if (handX - rightBarrier > 10) %safety
                scalingX = -springConst * 10;
            end
        else %left hand use
            scalingX = springConst * (rightBarrier - handX);
            if (handX - rightBarrier > 10) %safety
                scalingX = springConst * 10;
            end
        end
    else
        scalingX = 0;
    end
end

== matlab function KinarmSimonTask_260119/resultText/textMod ==
  data: textIn input; pickText input; textOut output
function textOut  = fcn(textIn, pickText)
%function modifies the trial result text with hardcoded text

textOut = textIn;
if (pickText == 1) %block starting text
    str1 = ['Keep your cursor inside the circle to begin'];
elseif (pickText == 2) %incorrect trials output
    str1 = ['Incorrect!'];
elseif (pickText == 3) %timed out trials output
    str1 = ['Too slow!'];
elseif (pickText == 4) %false start trials output
    str1 = ['Stay inside!'];
else %checks errors
    str1 = ['Error'];
end
textOut(1,15:(length(str1)+14))=uint16(str1);  %str in letters
